simulink model "W10B_FreqDesign"  (R2024b)
settings: Solver=ode45  StartTime=0.0  StopTime=t_end  MaxStep=1e-3  RelTol=1e-3
PreLoadFcn:
  | % W10B_FreqDesign 기본 파라미터 (모델을 열 때 자동 실행)
  | % 플랜트 G = 0.01/(0.005s^3+0.06s^2+0.1001s),  DC 모터 위치
  | % 제어기 C = 200*[(0.14416s+1)/(0.01433s+1)]^2  (강의노트 8-4 절)
  | defs = { 'numG',0.01 ; 'denG',[0.005 0.06 0.1001 0] ;
  |          'numC',200*conv([0.144164 1],[0.144164 1]) ;
  |          'denC',conv([0.014334 1],[0.014334 1]) ;
  |          'r_slope',0.2 ; 'tau',0.3 ;
  |          'Td',0.02 ;
  |          'u_lim',12 ; 'u_sat',12 ;
  |          't_end',4 };
  | for ii = 1:size(defs,1)
  |     if ~evalin('base', sprintf('exist(''%s'',''var'')', defs{ii,1}))
  |         assignin('base', defs{ii,1}, defs{ii,2});
  |     end
  | end
  | clear defs ii
values from neighbouring files (symbols this model uses):
  denC = conv([0.014334 1], [0.014334 1])    [W10B_06_run_simulink.m]
  denG = [0.005 0.06 0.1001 0]    [W10B_06_run_simulink.m]
  numC = 200*conv([0.144164 1], [0.144164 1])    [W10B_06_run_simulink.m]
  numG = 0.01    [W10B_06_run_simulink.m]
  r_slope = 0.2    [W10B_06_run_simulink.m]
  tau = 0.05    [W10B_02_pd_lead.m]    (also in W10B_06_run_simulink.m = 0.3)
  Td = 0.1    [W10B_02_pd_lead.m]    (also in W10B_06_run_simulink.m = 0.02)
  u_sat = 12    [W10B_06_run_simulink.m]
libraries: simulink x1
settings Model: Creator=admin  LastModifiedBy=admin
settings DataIOCC: OutputOption=SpecifiedOutputTimes  OutputTimes=0:0.001:t_end

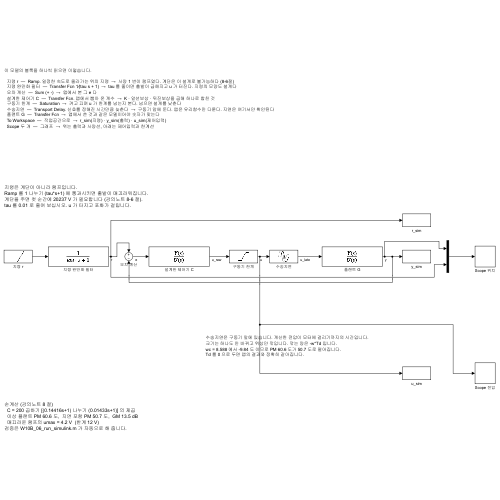
[thumbnail: Simulink's stored preview of the top-level diagram]
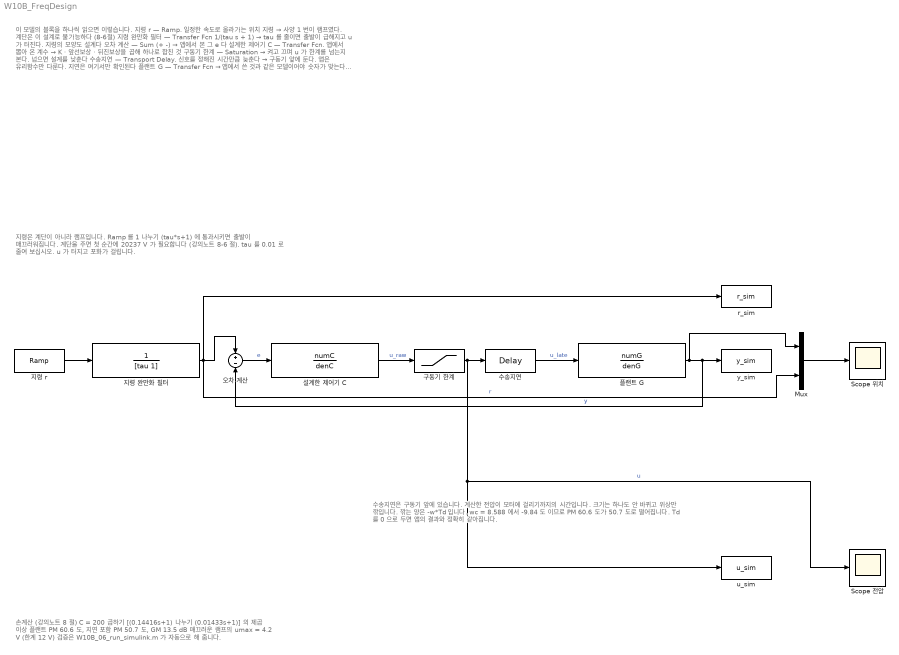
== system W10B_FreqDesign ==
  note: 지령은 계단이 아니라 램프입니다.
      | Ramp 를 1 나누기 (tau*s+1) 에 통과시키면 출발이 매끄러워집니다.
      | 계단을 주면 첫 순간에 20237 V 가 필요합니다 (강의노트 8-6 절).
      | tau 를 0.01 로 줄여 보십시오. u 가 터지고 포화가 걸립니다.
  note: 수송지연은 구동기 앞에 있습니다. 계산한 전압이 모터에 걸리기까지의 시간입니다.
      | 크기는 하나도 안 바뀌고 위상만 깎입니다. 깎는 양은 -w*Td 입니다.
      | wc = 8.588 에서 -9.84 도 이므로 PM 60.6 도가 50.7 도로 떨어집니다.
      | Td 를 0 으로 두면 앱의 결과와 정확히 같아집니다.
  note: 손계산 (강의노트 8 절)
      |   C = 200 곱하기 [(0.14416s+1) 나누기 (0.01433s+1)] 의 제곱
      |   이상 플랜트 PM 60.6 도,  지연 포함 PM 50.7 도,  GM 13.5 dB
      |   매끄러운 램프의 umax = 4.2 V  (한계 12 V)
      | 검증은 W10B_06_run_simulink.m 가 자동으로 해 줍니다.
  note: 이 모델의 블록을 하나씩 읽으면 이렇습니다.
      |
      |   지령 r  —  Ramp. 일정한 속도로 올라가는 위치 지령  →  사양 1 번이 램프였다. 계단은 이 설계로 불가능하다 (8-6절)
      |   지령 완만화 필터  —  Transfer Fcn 1∕(tau s + 1)  →  tau 를 줄이면 출발이 급해지고 u 가 터진다. 지령의 모양도 설계다
      |   오차 계산  —  Sum (+ -)  →  앱에서 본 그 e 다
      |   설계한 제어기 C  —  Transfer Fcn. 앱에서 뽑아 온 계수  →  K · 앞선보상 · 뒤진보상을 곱해 하나로 합친 것
      |   구동기 한계  —  Saturation  →  켜고 끄며 u 가 한계를 넘는지 본다. 넘으면 설계를 낮춘다
      |   수송지연  —  Transport Delay. 신호를 정해진 시간만큼 늦춘다  →  구동기 앞에 둔다. 앱은 유리함수만 다룬다. 지연은 여기서만 확인된다
      |   플랜트 G  —  Transfer Fcn  →  앱에서 쓴 것과 같은 모델이어야 숫자가 맞는다
      |   To Workspace  —  작업공간으로  →  r_sim(지령) · y_sim(출력) · u_sim(제어입력)
      |   Scope 두 개  —  그래프  →  위는 출력과 사양선, 아래는 제어입력과 한계선
  Mux : Mux  Inputs=2
  Scope 위치 : Scope
  Scope 전압 : Scope
  r_sim : ToWorkspace  VariableName=r_sim  SaveFormat=Timeseries  SampleTime=-1
  u_sim : ToWorkspace  VariableName=u_sim  SaveFormat=Timeseries  SampleTime=-1
  y_sim : ToWorkspace  VariableName=y_sim  SaveFormat=Timeseries  SampleTime=-1
  구동기 한계 : Saturate  UpperLimit=u_sat  LowerLimit=-u_sat
  설계한 제어기 C : TransferFcn  Numerator=numC  Denominator=denC
  수송지연 : TransportDelay  DelayTime=Td  BufferSize=16384
  오차 계산 : Sum  Inputs=+-
  지령 r : simulink/Sources/Ramp  slope=r_slope  start=0  InitialOutput=0
  지령 완만화 필터 : TransferFcn  Numerator=1  Denominator=[tau 1]
  플랜트 G : TransferFcn  Numerator=numG  Denominator=denG
  wires:
  지령 r/1 -> 지령 완만화 필터/1
  지령 완만화 필터/1 -> 오차 계산/1, Mux/2, r_sim/1  "r"
  오차 계산/1 -> 설계한 제어기 C/1  "e"
  설계한 제어기 C/1 -> 구동기 한계/1  "u_raw"
  구동기 한계/1 -> u_sim/1, Scope 전압/1, 수송지연/1  "u"
  수송지연/1 -> 플랜트 G/1  "u_late"
  플랜트 G/1 -> 오차 계산/2, y_sim/1, Mux/1  "y"
  Mux/1 -> Scope 위치/1
